simulink model "hdlcoder_fsm_eml"  (R2026a)
settings: Solver=FixedStepDiscrete  FixedStep=0.2  EnableMultiTasking=on
libraries: simulink x3
settings Model: ExtModeAutoUpdateStatusClock=off  Creator=The MathWorks, Inc.  LastModifiedBy=The MathWorks, Inc.
settings OptimizationCC: InitFltsAndDblsToZero=on
settings DebuggingCC: SaveWithParameterizedLinksMsg=none  UnderspecifiedInitializationDetection=Classic  SignalResolutionControl=TryResolveAllWithWarning  MultiTaskDSMMsg=warning  MultiTaskCondExecSysMsg=none
settings HardwareCC: ProdHWDeviceType=32-bit Generic  TargetHWDeviceType=32-bit Generic
settings GRTTargetCC: TargetFcnLib=ansi_tfl_tmw.mat  CombineOutputUpdateFcns=off  GRTInterface=on

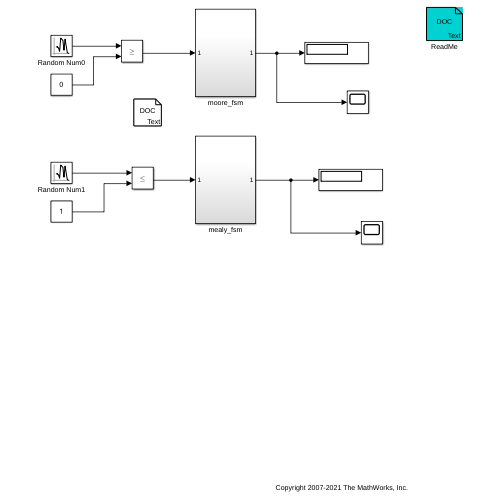
[thumbnail: Simulink's stored preview of the top-level diagram]
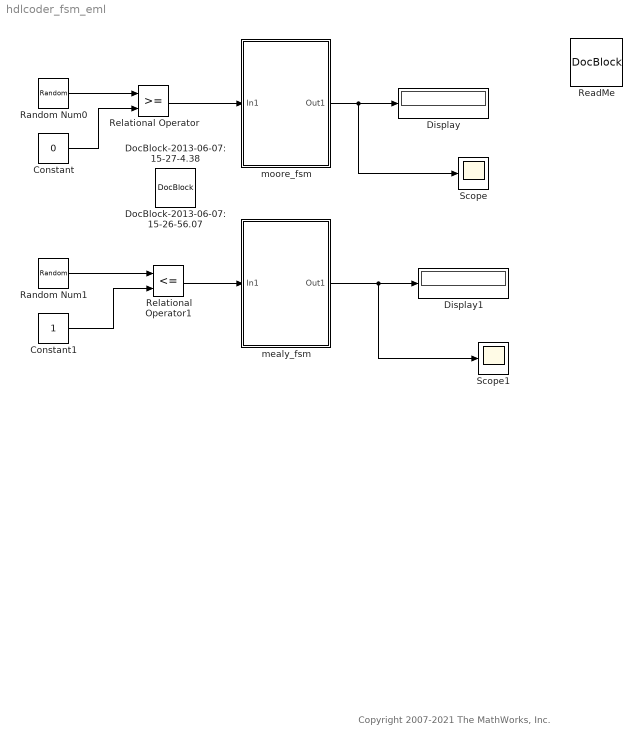
== system hdlcoder_fsm_eml ==
  note: Copyright 2007-2021 The MathWorks, Inc.
  Constant : Constant  Value=0
  Constant1 : Constant
  Display : Display
  Display1 : Display
  DocBlock-2013-06-07:15-26-56.07 : simulink/Model-Wide Utilities/DocBlock  DocumentType=Text
      content=|
      | Type your documentation here
  DocBlock-2013-06-07:15-27-4.38 : simulink/Model-Wide Utilities/DocBlock  DocumentType=Text
      content=|
      | Type your documentation here
  Random Num0 : RandomNumber  SampleTime=0
  Random Num1 : RandomNumber  SampleTime=0
  ReadMe : simulink/Model-Wide Utilities/DocBlock  DocumentType=Text
      content=|
      | A finite state machine is a representation of a reactive system.
      | In an event-driven system, the system makes a transition from one state
      | (mode) to another prescribed state, provided that the condition defining
      | the change is true.
      |
      | Stateflow is the best tool for modeling finite state machines.
      | It provides very sophisticated capabilities to build hierarchical and
      | parallel state machines, temporal logic and state entry/during/exit
      | actions etc.,
      |
      | However there are many Signal Processing and Communications applications
      | where in when writing a very data flow centric algorithms, there comes a
      | need to write a small controller embedded in the algorithm. This example
      | shows how to implement very simple mealy and more state machines using
      | Embedded MATLAB control flow constructs.
      |
      | Mealy: y = f(x,u)
      |  all actions are condition actions and outputs are function of state and input
      |
      | Moore: y = f(x)
      |  all actions are state actions and outputs are pure functions of state only
      |
      |
      | ============================================
      | To generate HDL code from the attached model
      | ============================================
      |
      | dut = 'hdlcoder_fsm_eml/moore_fsm';
      | tlang = 'vhdl';
      | tdir = ['hdlsrc' '_' tlang];
      |
      | makehdl(dut, 'targetlang', tlang, 'targetdir', tdir);
      | makehdltb(dut, 'targetlang', tlang, 'targetdir', tdir);
      |
      |
      | dut = 'hdlcoder_fsm_eml/mealy_fsm';
      | tlang = 'verilog';
      | tdir = ['hdlsrc' '_' tlang];
      |
      | makehdl(dut, 'targetlang', tlang, 'targetdir', tdir);
      | makehdltb(dut, 'targetlang', tlang, 'targetdir', tdir);
  Relational Operator : RelationalOperator  OutDataTypeStr=boolean  InputSameDT=off
  Relational Operator1 : RelationalOperator  Operator=<=  OutDataTypeStr=boolean  InputSameDT=off
  Scope : Scope
  Scope1 : Scope
  mealy_fsm : Subsystem
  moore_fsm : Subsystem
  wires:
  Random Num0/1 -> Relational Operator/1
  Constant/1 -> Relational Operator/2
  Relational Operator/1 -> moore_fsm/1(In1)
  moore_fsm/1(Out1) -> Display/1, Scope/1
  mealy_fsm/1(Out1) -> Display1/1, Scope1/1
  Random Num1/1 -> Relational Operator1/1
  Constant1/1 -> Relational Operator1/2
  Relational Operator1/1 -> mealy_fsm/1(In1)

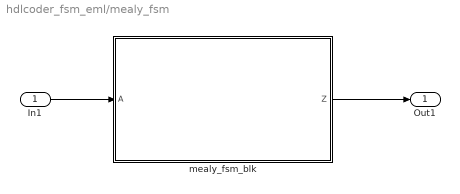
== system hdlcoder_fsm_eml/mealy_fsm ==
  In1 : Inport
  mealy_fsm_blk : MATLAB Function  TreatAsAtomicUnit=on
  Out1 : Outport
  wires:
  In1/1 -> mealy_fsm_blk/1(A)
  mealy_fsm_blk/1(Z) -> Out1/1

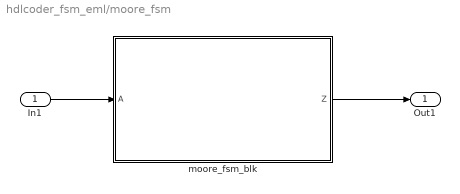
== system hdlcoder_fsm_eml/moore_fsm ==
  In1 : Inport
  moore_fsm_blk : MATLAB Function  TreatAsAtomicUnit=on
  Out1 : Outport
  wires:
  moore_fsm_blk/1(Z) -> Out1/1
  In1/1 -> moore_fsm_blk/1(A)

== matlab function hdlcoder_fsm_eml/moore_fsm/moore_fsm_blk ==
  settings: fimath=|
      | fimath(...
      | 'RoundMode', 'nearest',...
      | 'OverflowMode', 'saturate',...
      | 'ProductMode', 'FullPrecision', 'ProductWordLength', 128,...
      | 'SumMode', 'FullPrecision', 'SumWordLength', 128,...
      | 'CastBeforeSum', true)
  data: A input boolean; Z output boolean size=1
function Z = moore_fsm(A)
% Moore State Machine

% y = f(x) : 
% all actions are state actions and 
% outputs are pure functions of state only 

% using persistent keyword to model state registers in hardware
persistent moore_state_reg;
if isempty(moore_state_reg)
    moore_state_reg = fi(0, 0, 2, 0);   
end

S1 = 0;
S2 = 1;
S3 = 2;
S4 = 3;

% switch to new state based on the value state register
switch (moore_state_reg)
    
    case S1
        
        % value of output 'Z' depends both only on state and not on inputs
        Z = true;
        
        % decide next state value based on inputs
        if (~A)
            moore_state_reg(1) = S1;
        else
            moore_state_reg(1) = S2;
        end
        
    case S2
        
        Z = false;
        
        if (~A)
            moore_state_reg(1) = S1;
        else
            moore_state_reg(1) = S2;
        end
        
    case S3
        
        Z = false;
        
        if (~A)
            moore_state_reg(1) = S2;
        else
            moore_state_reg(1) = S3;
        end
        
    case S4
        
        Z = true;
        if (~A)
            moore_state_reg(1) = S1;
        else
            moore_state_reg(1) = S3;
        end
    otherwise
        Z = false;
end

== matlab function hdlcoder_fsm_eml/mealy_fsm/mealy_fsm_blk ==
  settings: fimath=|
      | fimath(...
      | 'RoundMode', 'nearest',...
      | 'OverflowMode', 'saturate',...
      | 'ProductMode', 'FullPrecision', 'ProductWordLength', 128,...
      | 'SumMode', 'FullPrecision', 'SumWordLength', 128,...
      | 'CastBeforeSum', true)
  data: A input boolean; Z output boolean size=1
function Z = mealy_fsm(A)
% Mealy State Machine

% y = f(x,u) : 
% all actions are condition actions and 
% outputs are function of state and input 

persistent mealy_state_reg;
if isempty(mealy_state_reg)
    mealy_state_reg = fi(0, 0, 2, 0);   
end

S1 = 0;
S2 = 1;
S3 = 2;
S4 = 3;

% switch to new state based on the value state register
switch (mealy_state_reg) 
    
    case S1
        
        % value of output 'Z' depends both on state and inputs
        if (A)
            Z = true;
            mealy_state_reg(1) = S1;
        else
            Z = false;            
            mealy_state_reg(1) = S2;
        end
        
    case S2
        
        if (A)
            Z = false;
            mealy_state_reg(1) = S1;
        else
            Z = true;
            mealy_state_reg(1) = S2;
        end
        
    case S3
        
        if (A)
            Z = false;            
            mealy_state_reg(1) = S2;
        else
            Z = true;            
            mealy_state_reg(1) = S3;
        end
        
    case S4
        
        if (A)
            Z = true;
            mealy_state_reg(1) = S1;
        else
            Z = false;            
            mealy_state_reg(1) = S3;
        end        
        
    otherwise
        
        Z = false;
end
